simulink model "Z1"  (R2023b)
settings: Solver=VariableStepAuto  StartTime=0.0  StopTime=20  RelTol=1e-3
settings Model: Creator=Liu  LastModifiedBy=Liu

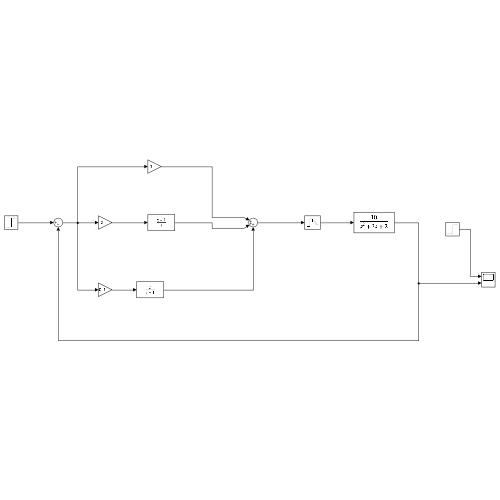
[thumbnail: Simulink's stored preview of the top-level diagram]
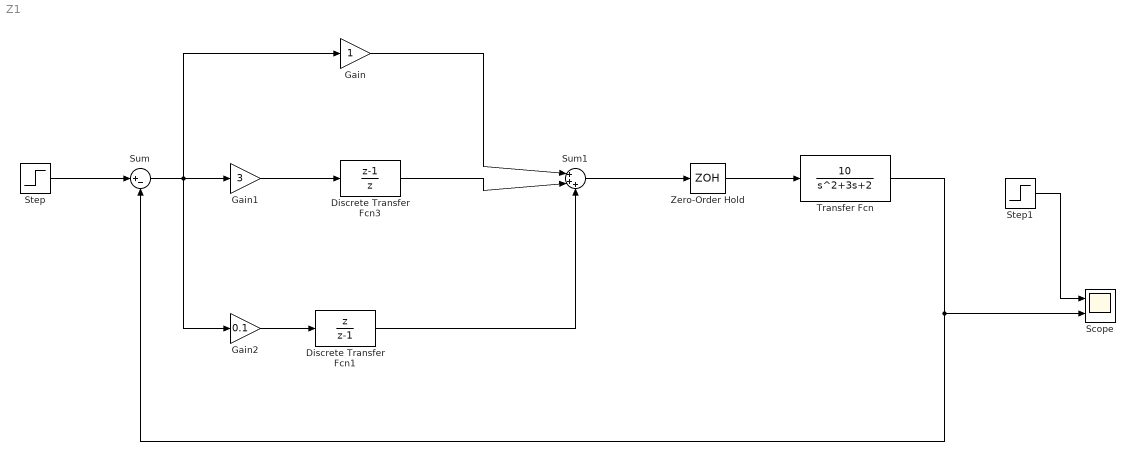
== system Z1 ==
  Discrete Transfer Fcn1 : DiscreteTransferFcn  Numerator=[1 0]  Denominator=[1 -1]
  Discrete Transfer Fcn3 : DiscreteTransferFcn  Numerator=[1 -1]  Denominator=[1 0]
  Gain : Gain
  Gain1 : Gain  Gain=3
  Gain2 : Gain  Gain=0.1
  Scope : Scope  NumInputPorts=2
  Step : Step  SampleTime=0
  Step1 : Step  SampleTime=0
  Sum : Sum  Inputs=|+-
  Sum1 : Sum  Inputs=|+++
  Transfer Fcn : TransferFcn  Numerator=[0 10]  Denominator=[1 3 2]
  Zero-Order Hold : ZeroOrderHold  SampleTime=0.1
  wires:
  Step/1 -> Sum/1
  Sum/1 -> Gain/1, Gain2/1, Gain1/1
  Gain2/1 -> Discrete Transfer Fcn1/1
  Gain1/1 -> Discrete Transfer Fcn3/1
  Gain/1 -> Sum1/1
  Sum1/1 -> Zero-Order Hold/1
  Transfer Fcn/1 -> Sum/2, Scope/2
  Step1/1 -> Scope/1
  Zero-Order Hold/1 -> Transfer Fcn/1
  Discrete Transfer Fcn3/1 -> Sum1/2
  Discrete Transfer Fcn1/1 -> Sum1/3
